simulink model "model_arbore"  (R2026a)
settings: Solver=ode45  StopTime=Tsim  MaxStep=2e-5  RelTol=1e-8  AbsTol=1e-8
model workspace (MAT data in the model file):
  J0 = 0.00520010634034
  Tff_tab = [0.94926679139 0.709220063818 0.468754259873 0.227887723987 -0.0133611334008 -0.254973839716 -0.496931864131 -0.739216621458 -0.981809476051 -1.22469174571 -1.46784470561 -1.71124959218 ... (3601 elements, 3601x1)]
  Tg_tab = [0 0.240046727572 0.480512531517 0.721379067403 0.962627924791 1.20424063111 1.44619865552 1.68848341285 1.93107626744 2.1739585371 2.417111497 2.66051638357 ... (3601 elements, 3601x1)]
  Tmean = 1.986525
  Tsim = 1
  d2x_tab = [0.0340005681818 0.0340004874439 0.0340002452305 0.0339998415432 0.0339992763847 0.0339985497585 0.0339976616694 0.0339966121229 0.0339954011259 0.033994028686 0.0339924948122 0.0339907995141 ... (3601 elements, 3601x1)]
  dx_tab = [0 5.93421392607e-05 0.000118683996693 0.00017802529047 0.00023736573877 0.000296705059774 0.000356042971673 0.000415379192664 0.000474713440958 0.000534045434777 0.000593374892357 0.000652701531952 ... (3601 elements, 3601x1)]
  m_rec = 0.255
  tau = 0.0005
  th_tab = [0 0.00174532925199 0.00349065850399 0.00523598775598 0.00698131700798 0.00872664625997 0.010471975512 0.012217304764 0.013962634016 0.0157079632679 0.0174532925199 0.0191986217719 ... (3601 elements, 3601x1)]
  w0 = 157.079632679
  w_ref = 157.079632679
Description:
  | Dinamica arborelui cotit cu volant activ (MIL-1). Generat de m01_model_arbore.m; datele vin din parametri.m. Nu se editează de mână.
settings Model: Creator=Darian  LastModifiedBy=Darian

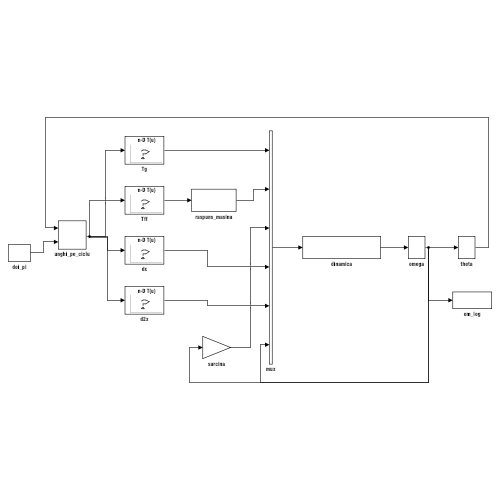
[thumbnail: Simulink's stored preview of the top-level diagram]
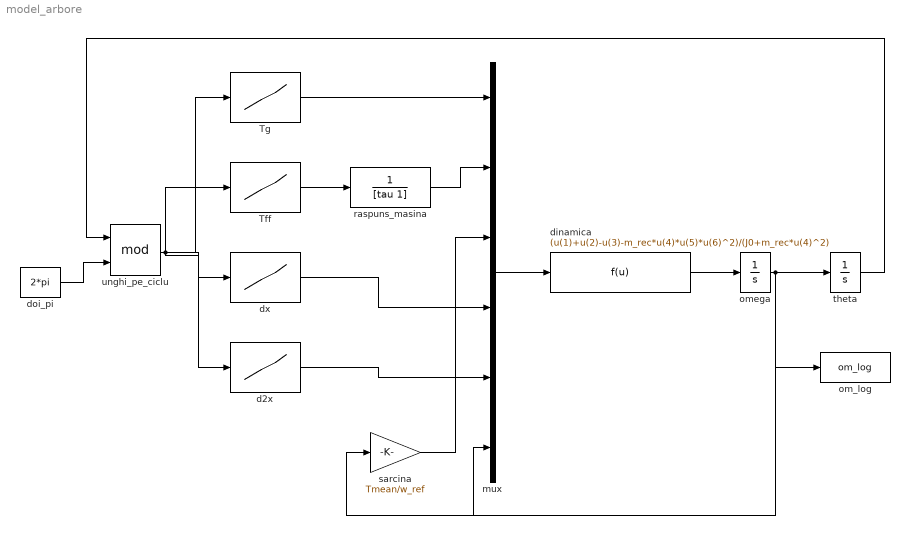
== system model_arbore ==
  Tff : Lookup_n-D  NumberOfTableDimensions=1  BreakpointsForDimension1=th_tab  Table=Tff_tab  InternalRulePriority=Speed  RndMeth=Simplest
  Tg : Lookup_n-D  NumberOfTableDimensions=1  BreakpointsForDimension1=th_tab  Table=Tg_tab  InternalRulePriority=Speed  RndMeth=Simplest
  d2x : Lookup_n-D  NumberOfTableDimensions=1  BreakpointsForDimension1=th_tab  Table=d2x_tab  InternalRulePriority=Speed  RndMeth=Simplest
  dinamica : Fcn  Expr=(u(1)+u(2)-u(3)-m_rec*u(4)*u(5)*u(6)^2)/(J0+m_rec*u(4)^2)
  doi_pi : Constant  Value=2*pi
  dx : Lookup_n-D  NumberOfTableDimensions=1  BreakpointsForDimension1=th_tab  Table=dx_tab  InternalRulePriority=Speed  RndMeth=Simplest
  mux : Mux  Inputs=6
  om_log : ToWorkspace  VariableName=om_log  SaveFormat=Timeseries  SampleTime=-1
  omega : Integrator  InitialCondition=w0
  raspuns_masina : TransferFcn  Numerator=1  Denominator=[tau 1]
  sarcina : Gain  Gain=Tmean/w_ref
  theta : Integrator
  unghi_pe_ciclu : Math  Operator=mod
  wires:
  dinamica/1 -> omega/1
  omega/1 -> theta/1, sarcina/1, mux/6, om_log/1
  theta/1 -> unghi_pe_ciclu/1
  doi_pi/1 -> unghi_pe_ciclu/2
  unghi_pe_ciclu/1 -> Tg/1, Tff/1, dx/1, d2x/1
  Tff/1 -> raspuns_masina/1
  Tg/1 -> mux/1
  raspuns_masina/1 -> mux/2
  sarcina/1 -> mux/3
  dx/1 -> mux/4
  d2x/1 -> mux/5
  mux/1 -> dinamica/1
